simulink model "vienna_rectifier"  (R2026b)
settings: Solver=ode23tb  StopTime=param.sim.simlength  FixedStep=param.glb_time.tc  MaxStep=param.glb_time.tc
values from neighbouring files (symbols this model uses):
  param = struct()    [init_model.m]
undefined symbols (not defined in the file or in its folder): magnitude
libraries: fl_lib x42, nesl_utility x28, discrete_time_low_pass_filter x5, single_phase_transformer_lib x3, threephase_inductor_lib x1, dclink_for_three_levels x1, vienna_rectifier_ideal_switch_based_model x1, three_phase_three_levels_PWM_modulator x1, three_phase_voltage_with_frt_emulator x1
(part 2 of 4)

== system vienna_rectifier/grid/grid_emulator/3ph_Dyg ==
  Electrical Reference1 : fl_lib/Electrical/Electrical Elements/Electrical Reference
  ph1 : single_phase_transformer_lib/single phase transformer  Lm=param.grid.emu.trafo.Lm1 H  n1=param.grid.emu.trafo.n1  n2=param.grid.emu.trafo.n2  Rd1=param.grid.emu.trafo.Rd1 Ohm  Rd2=param.grid.emu.trafo.Rd2 Ohm  Ld1=param.grid.emu.trafo.Ld1 H  Ld2=param.grid.emu.trafo.Ld2 H  Rfe=param.grid.emu.trafo.Rfe1 Ohm  phi_specify=off  phi_priority=None  phi=0 V*s  phi_nominal_specify=off  phi_nominal_value=1  phi_nominal_unit=V*s  i1_specify=off  i1_priority=None  i1=0 A  i1_nominal_specify=off  i1_nominal_value=1  i1_nominal_unit=A  i2_specify=off  i2_priority=None  i2=0 A  i2_nominal_specify=off  i2_nominal_value=1  i2_nominal_unit=A  ife_specify=off  ife_priority=None  ife=0 A  ife_nominal_specify=off  ife_nominal_value=1  ife_nominal_unit=A  u1_specify=off  u1_priority=None  u1=0 V  u1_nominal_specify=off  u1_nominal_value=1  u1_nominal_unit=V  u2_specify=off  u2_priority=None  u2=0 V  u2_nominal_specify=off  u2_nominal_value=1  u2_nominal_unit=V
  ph2 : single_phase_transformer_lib/single phase transformer  Lm=param.grid.emu.trafo.Lm1 H  n1=param.grid.emu.trafo.n1  n2=param.grid.emu.trafo.n2  Rd1=param.grid.emu.trafo.Rd1 Ohm  Rd2=param.grid.emu.trafo.Rd2 Ohm  Ld1=param.grid.emu.trafo.Ld1 H  Ld2=param.grid.emu.trafo.Ld2 H  Rfe=param.grid.emu.trafo.Rfe1 Ohm  phi_specify=off  phi_priority=None  phi=0 V*s  phi_nominal_specify=off  phi_nominal_value=1  phi_nominal_unit=V*s  i1_specify=off  i1_priority=None  i1=0 A  i1_nominal_specify=off  i1_nominal_value=1  i1_nominal_unit=A  i2_specify=off  i2_priority=None  i2=0 A  i2_nominal_specify=off  i2_nominal_value=1  i2_nominal_unit=A  ife_specify=off  ife_priority=None  ife=0 A  ife_nominal_specify=off  ife_nominal_value=1  ife_nominal_unit=A  u1_specify=off  u1_priority=None  u1=0 V  u1_nominal_specify=off  u1_nominal_value=1  u1_nominal_unit=V  u2_specify=off  u2_priority=None  u2=0 V  u2_nominal_specify=off  u2_nominal_value=1  u2_nominal_unit=V
  ph3 : single_phase_transformer_lib/single phase transformer  Lm=param.grid.emu.trafo.Lm1 H  n1=param.grid.emu.trafo.n1  n2=param.grid.emu.trafo.n2  Rd1=param.grid.emu.trafo.Rd1 Ohm  Rd2=param.grid.emu.trafo.Rd2 Ohm  Ld1=param.grid.emu.trafo.Ld1 H  Ld2=param.grid.emu.trafo.Ld2 H  Rfe=param.grid.emu.trafo.Rfe1 Ohm  phi_specify=off  phi_priority=None  phi=0 V*s  phi_nominal_specify=off  phi_nominal_value=1  phi_nominal_unit=V*s  i1_specify=off  i1_priority=None  i1=0 A  i1_nominal_specify=off  i1_nominal_value=1  i1_nominal_unit=A  i2_specify=off  i2_priority=None  i2=0 A  i2_nominal_specify=off  i2_nominal_value=1  i2_nominal_unit=A  ife_specify=off  ife_priority=None  ife=0 A  ife_nominal_specify=off  ife_nominal_value=1  ife_nominal_unit=A  u1_specify=off  u1_priority=None  u1=0 V  u1_nominal_specify=off  u1_nominal_value=1  u1_nominal_unit=V  u2_specify=off  u2_priority=None  u2=0 V  u2_nominal_specify=off  u2_nominal_value=1  u2_nominal_unit=V
  ua : PMIOPort  Side=Right
  ub : PMIOPort  Port=2  Side=Right
  uc : PMIOPort  Port=3  Side=Right
  Ua : PMIOPort  Port=4  Side=Left
  Ub : PMIOPort  Port=5  Side=Left
  Uc : PMIOPort  Port=6  Side=Left
  connections:
  Electrical Reference1/LConn1 -- ph3/RConn2 -- ph2/RConn2 -- ph1/RConn2
  ph3/RConn1 -- uc/RConn1
  ph1/LConn1 -- ph3/LConn2 -- Ua/RConn1
  ph1/RConn1 -- ua/RConn1
  ph2/RConn1 -- ub/RConn1
  ph1/LConn2 -- ph2/LConn1 -- Ub/RConn1
  Uc/RConn1 -- ph3/LConn1 -- ph2/LConn2

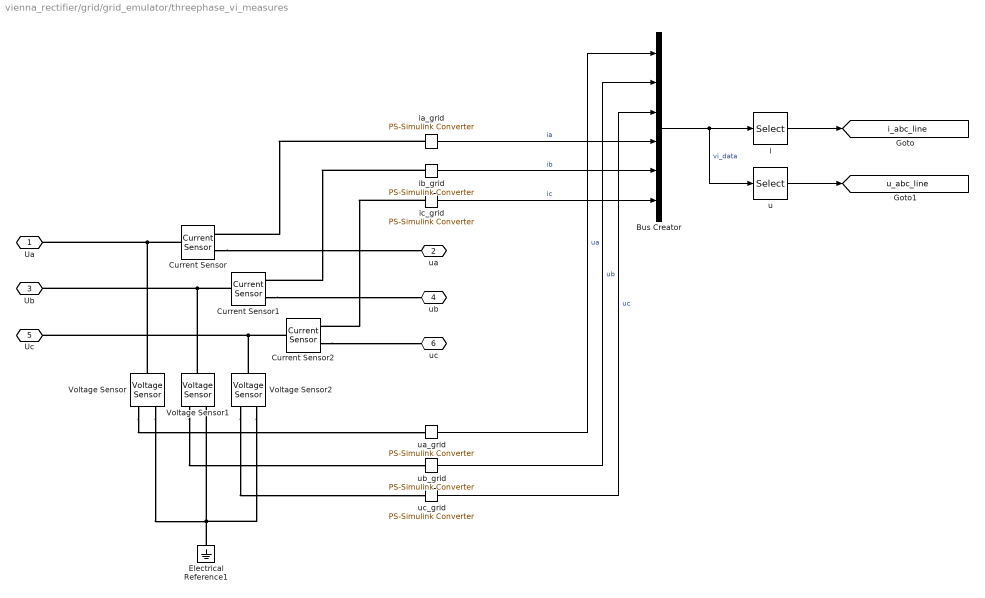
== system vienna_rectifier/grid/grid_emulator/threephase_vi_measures ==
  Bus Creator : BusCreator  Inputs=6
  Current Sensor : fl_lib/Electrical/Electrical Sensors/Current Sensor
  Current Sensor1 : fl_lib/Electrical/Electrical Sensors/Current Sensor
  Current Sensor2 : fl_lib/Electrical/Electrical Sensors/Current Sensor
  Electrical Reference1 : fl_lib/Electrical/Electrical Elements/Electrical Reference
  Voltage Sensor : fl_lib/Electrical/Electrical Sensors/Voltage Sensor
  Voltage Sensor1 : fl_lib/Electrical/Electrical Sensors/Voltage Sensor
  Voltage Sensor2 : fl_lib/Electrical/Electrical Sensors/Voltage Sensor
  i : Selector  InputPortWidth=6  IndexOptions=Index vector (dialog)  Indices=[4 5 6]  OutputSizes=1  RuntimeRangeChecks=off
  ia_grid : nesl_utility/PS-Simulink Converter  PhysicalDomain=network_engine_domain  SubClassName=ps_output  LeftPortType=input  RightPortType=output  PseudoPeriodic=off  Frequencies=[]  VectorFormat=1-D array  Unit=A  AffineConversion=off
  ib_grid : nesl_utility/PS-Simulink Converter  PhysicalDomain=network_engine_domain  SubClassName=ps_output  LeftPortType=input  RightPortType=output  PseudoPeriodic=off  Frequencies=[]  VectorFormat=1-D array  Unit=A  AffineConversion=off
  ic_grid : nesl_utility/PS-Simulink Converter  PhysicalDomain=network_engine_domain  SubClassName=ps_output  LeftPortType=input  RightPortType=output  PseudoPeriodic=off  Frequencies=[]  VectorFormat=1-D array  Unit=A  AffineConversion=off
  u : Selector  InputPortWidth=6  IndexOptions=Index vector (dialog)  Indices=[1 2 3]  OutputSizes=1  RuntimeRangeChecks=off
  ua_grid : nesl_utility/PS-Simulink Converter  PhysicalDomain=network_engine_domain  SubClassName=ps_output  LeftPortType=input  RightPortType=output  PseudoPeriodic=off  Frequencies=[]  VectorFormat=1-D array  Unit=V  AffineConversion=off
  ub_grid : nesl_utility/PS-Simulink Converter  PhysicalDomain=network_engine_domain  SubClassName=ps_output  LeftPortType=input  RightPortType=output  PseudoPeriodic=off  Frequencies=[]  VectorFormat=1-D array  Unit=V  AffineConversion=off
  uc_grid : nesl_utility/PS-Simulink Converter  PhysicalDomain=network_engine_domain  SubClassName=ps_output  LeftPortType=input  RightPortType=output  PseudoPeriodic=off  Frequencies=[]  VectorFormat=1-D array  Unit=V  AffineConversion=off
  Ua : PMIOPort  Side=Left
  ua : PMIOPort  Port=2  Side=Right
  Ub : PMIOPort  Port=3  Side=Left
  ub : PMIOPort  Port=4  Side=Right
  Uc : PMIOPort  Port=5  Side=Left
  uc : PMIOPort  Port=6  Side=Right
  tag scope: i_abc_line=global, u_abc_line=global
  wires:
  Bus Creator/1 -> i/1, u/1  "vi_data"
  ib_grid/1 -> Bus Creator/5  "ib"
  ia_grid/1 -> Bus Creator/4  "ia"
  ic_grid/1 -> Bus Creator/6  "ic"
  ua_grid/1 -> Bus Creator/1  "ua"
  ub_grid/1 -> Bus Creator/2  "ub"
  uc_grid/1 -> Bus Creator/3  "uc"
  i/1 -> [i_abc_line]
  u/1 -> [u_abc_line]
  connections:
  Current Sensor1/LConn1 -- Ub/RConn1 -- Voltage Sensor1/LConn1
  Electrical Reference1/LConn1 -- Voltage Sensor/RConn2 -- Voltage Sensor2/RConn2 -- Voltage Sensor1/RConn2
  Voltage Sensor/RConn1 -- ua_grid/LConn1
  Current Sensor/RConn2 -- ua/RConn1
  Voltage Sensor1/RConn1 -- ub_grid/LConn1
  Voltage Sensor2/LConn1 -- Current Sensor2/LConn1 -- Uc/RConn1
  Current Sensor/LConn1 -- Ua/RConn1 -- Voltage Sensor/LConn1
  Current Sensor1/RConn2 -- ub/RConn1
  Voltage Sensor2/RConn1 -- uc_grid/LConn1
  ib_grid/LConn1 -- Current Sensor1/RConn1
  ia_grid/LConn1 -- Current Sensor/RConn1
  ic_grid/LConn1 -- Current Sensor2/RConn1
  Current Sensor2/RConn2 -- uc/RConn1

== system vienna_rectifier/afe_dq_mod1/AFE_control/afe_control/acquisitions ==
  ug_abc_pu : Inport
  udc_pu : Inport  Port=2
  ig_abc_pu : Inport  Port=3
  is_abc_pu : Inport  Port=4
  master_time : Inport  Port=5
  grid_phase : Inport  Port=6
  Terminator : Terminator
  grid_phase_acquisition : Subsystem
  ig afe quantizzation and one step delay : Subsystem
  is afe quantizzation and one step delay : Subsystem
  phase_compensation_1 : Subsystem
  udc_acquisition : Subsystem
  ug afe quantizzation and one step delay : Subsystem
  AFE1_local_time_corr : Outport
  tag scope: grid_emulator_phase=scoped, igd_abc_pu=scoped, isd_abc_pu=scoped, udcd_pu_afe=scoped, ugd_abc_pu=scoped
  wires:
  grid_phase/1 -> grid_phase_acquisition/1(grid_phase)
  grid_phase_acquisition/1(grid_phased) -> [grid_emulator_phase]
  udc_acquisition/1(udcd_pu) -> [udcd_pu_afe]
  ig_abc_pu/1 -> ig afe quantizzation and one step delay/1(ig_abc_pu)
  ug_abc_pu/1 -> ug afe quantizzation and one step delay/1(ug_abc_pu)
  [udcd_pu_afe] -> Terminator/1
  phase_compensation_1/1(y) -> AFE1_local_time_corr/1
  is_abc_pu/1 -> is afe quantizzation and one step delay/1(is_abc_pu)
  master_time/1 -> phase_compensation_1/2(master_time)
  udc_pu/1 -> udc_acquisition/1(udc_pu)
  ig afe quantizzation and one step delay/1(igd_abc_pu) -> [igd_abc_pu]
  [local_time] -> phase_compensation_1/1(local_time)
  is afe quantizzation and one step delay/1(isd_abc_pu) -> [isd_abc_pu]
  ug afe quantizzation and one step delay/1(ugd_abc_pu) -> [ugd_abc_pu]

== system vienna_rectifier/afe_dq_mod1/AFE_control/afe_control/current_ctrl ==
  i_xi_ref : Inport
  Constant : Constant  Value=0
  Demux : Demux  Outputs=3
  current_transformation : Subsystem
  dq_vector_pi : Subsystem
  xi_eta_to_alpha_beta : MATLAB Function  TreatAsAtomicUnit=on
  zero_current_ctrl : Subsystem
  uabg : Outport  VectorParamsAs1DForOutWhenUnconnected=off
  wires:
  Demux/1 -> current_transformation/1(is_a_pu)  "is_a"
  Demux/2 -> current_transformation/2(is_b_pu)  "is_b"
  Demux/3 -> current_transformation/3(is_c_pu)  "is_c"
  [isd_abc_pu] -> Demux/1
  [phase_grid_pll] -> xi_eta_to_alpha_beta/3(phase)
  [id_xi_pu] -> dq_vector_pi/1(id)
  [id_eta_pu] -> dq_vector_pi/3(iq)
  i_xi_ref/1 -> dq_vector_pi/2(id_ref)
  Constant/1 -> dq_vector_pi/4(iq_ref)
  zero_current_ctrl/1(uabg_ctrl_out) -> uabg/1
  dq_vector_pi/1(md_sat) -> xi_eta_to_alpha_beta/1(xi)
  dq_vector_pi/2(mq_sat) -> xi_eta_to_alpha_beta/2(eta)
  xi_eta_to_alpha_beta/1(alpha) -> zero_current_ctrl/1(ualpha_ctrl_afe)
  xi_eta_to_alpha_beta/2(beta) -> zero_current_ctrl/2(ubeta_ctrl_afe)

== system vienna_rectifier/afe_dq_mod1/AFE_control/afe_control/data_to_worspace_module_1 ==
  Bus Creator : BusCreator  Inputs=3
  dq_pll : Subsystem
  pwr_meter : Subsystem
  m : Outport
  wires:
  Bus Creator/1 -> m/1
  pwr_meter/1(m_pwr_meter) -> Bus Creator/1  "pwr_meter"
  dq_pll/1(dqPLLs) -> Bus Creator/2  "dq_pll"
  [local_time] -> Bus Creator/3  "local_time"

== system vienna_rectifier/afe_dq_mod1/AFE_control/afe_control/grid_voltage_phase_lock_loops ==
  ug_abc_pu : Inport
  DDSRF-PLL : Subsystem
  tag scope: omega_grid_pll_pu=scoped, phase_grid_pll=scoped
  wires:
  ug_abc_pu/1 -> DDSRF-PLL/1(ug_abc_pu)
  DDSRF-PLL/1(gamma_grid_ddsrf_pll) -> [phase_grid_pll]
  DDSRF-PLL/2(omega_grid_ddsrf_pll) -> [omega_grid_pll_pu]

== system vienna_rectifier/afe_dq_mod1/AFE_control/afe_control/space_vector ==
  uab_out : Inport
  Bus Creator : BusCreator  Inputs=3
  Bus Selector : BusSelector  OutputSignals=da,db,dc
  Bus Selector1 : BusSelector  OutputSignals=ualpha_ctrl_afe,ubeta_ctrl_afe,ugamma_ctrl_afe
  C Caller : CCaller  FunctionName=sv_pwm_cm_process_simulink  PortSpecificationStruct="%)30     .    B H   8    (     @         %    \"     8    !     0         %  0 \"0    $    _    07)G3F%M90  4&]R=$YA;64 4V-O<&4     26YD97@     5'EP90      4VEZ90      27-';&]B86P   X    P    !@    @    $          4    (     0    ,    !         !   P!O=70 #@   #     &    \"     0         !0    @    !     P    $         $  # &]U=  .    .     8    (    !          %    \"     $    &     0         0   ...(+3252 chars)"
  Constant : Constant  Value=param.glb_time.ts_afe
  Constant1 : Constant
  Data Type Conversion1 : DataTypeConversion  OutDataTypeStr=double  SaturateOnIntegerOverflow=off  RndMeth=Floor
  Data Type Conversion{4,15..16,18} (4 alike) : DataTypeConversion  OutDataTypeStr=single  SaturateOnIntegerOverflow=off  RndMeth=Floor
  Data Type Conversion17 : DataTypeConversion  OutDataTypeStr=uint32  SaturateOnIntegerOverflow=off  RndMeth=Floor
  Data Type Conversion2 : DataTypeConversion  OutDataTypeStr=double  SaturateOnIntegerOverflow=off  RndMeth=Floor
  Data Type Conversion3 : DataTypeConversion  OutDataTypeStr=double  SaturateOnIntegerOverflow=off  RndMeth=Floor
  Gain1 : Gain  Gain=sqrt(3)/2
  Gain2 : Gain  Gain=sqrt(3)/2
  Gain3 : Gain  Gain=param.afe.behav.u_cm_comp_mod1
  duvw : Outport
  wires:
  Data Type Conversion15/1 -> C Caller/2
  Bus Selector/2 -> Data Type Conversion2/1  "<db>"
  Data Type Conversion18/1 -> C Caller/1
  C Caller/1 -> Bus Selector/1
  Bus Creator/1 -> duvw/1
  Data Type Conversion1/1 -> Bus Creator/1  "du(k)"
  Bus Selector1/2 -> Gain2/1  "<ubeta_ctrl_afe>"
  Bus Selector/3 -> Data Type Conversion3/1  "<dc>"
  Bus Selector1/1 -> Gain1/1  "<ualpha_ctrl_afe>"
  Data Type Conversion2/1 -> Bus Creator/2  "dv(k)"
  Gain2/1 -> Data Type Conversion15/1
  Bus Selector/1 -> Data Type Conversion1/1  "<da>"
  Gain1/1 -> Data Type Conversion18/1
  Data Type Conversion3/1 -> Bus Creator/3  "dw(k)"
  Constant/1 -> Data Type Conversion16/1
  uab_out/1 -> Bus Selector1/1
  Constant1/1 -> Data Type Conversion17/1
  Data Type Conversion16/1 -> C Caller/4
  Data Type Conversion17/1 -> C Caller/5
  Bus Selector1/3 -> Gain3/1  "<ugamma_ctrl_afe>"
  Gain3/1 -> Data Type Conversion4/1
  Data Type Conversion4/1 -> C Caller/3

== system vienna_rectifier/afe_dq_mod1/AFE_control/afe_control/udc_ctrl ==
  udc_pu : Inport
  1/Ti : Gain  Gain=param.afe.ctrl.kp_udc_ctrl  SaturateOnIntegerOverflow=on  OutDataTypeStr=Inherit: Same as input  ParamDataTypeStr=Inherit: Same as input
  Constant : Constant  Value=0
  Gain : Gain
  Saturation : Saturate  UpperLimit=param.afe.ctrl.ixi_pos_ref_lim  LowerLimit=-param.afe.ctrl.ixi_pos_ref_lim
  Sum1 : Sum  Inputs=+++  SaturateOnIntegerOverflow=on
  Sum2 : Sum  Inputs=-+  SaturateOnIntegerOverflow=on
  Sum3 : Sum  Inputs=-+  SaturateOnIntegerOverflow=on
  Switch : Switch  Criteria=u2 > Threshold  SaturateOnIntegerOverflow=off  InputSameDT=off
  To Workspace1 : ToWorkspace  VariableName=udc_pu_sim_mod1  SampleTime=-1
      settings: MaxDataPoints=param.glb_time.Ns_afe
  To Workspace3 : ToWorkspace  VariableName=udc_pu_ref_sim_mod1  SampleTime=-1
      settings: MaxDataPoints=param.glb_time.Ns_afe
  Unit Delay4 : UnitDelay  SampleTime=-1
  discrete-time-low-pass-filter1 : discrete_time_low_pass_filter/discrete-time-low-pass-filter  tau=20e-3  ts=param.glb_time.ts_afe
  kp : Gain  Gain=param.afe.ctrl.ki_udc_ctrl*param.glb_time.ts_afe  SaturateOnIntegerOverflow=on  OutDataTypeStr=Inherit: Same as input  ParamDataTypeStr=Inherit: Same as input
  pwr_lim_enable : Constant  Value=param.afe.behav.pwr_lim_enable
  udc_norm_ref : Step  Time=1e-3  FinalValue=param.afe.ctrl.udc_norm_ref
  udc_tracking : Scope  NumInputPorts=3
      settings: ActiveDisplayYMinimum=-0.20844726562499993  ActiveDisplayYMaximum=1.856494140625  DataLoggingVariableName=ScopeData8
  i_xi_ref : Outport
  wires:
  1/Ti/1 -> Sum1/1, Sum3/1
  kp/1 -> Sum1/2
  Sum3/1 -> Unit Delay4/1
  Unit Delay4/1 -> Sum1/3
  udc_norm_ref/1 -> discrete-time-low-pass-filter1/1
  udc_pu/1 -> Sum2/1, To Workspace1/1, udc_tracking/2  "udc_pu"
  Sum2/1 -> kp/1, 1/Ti/1
  Sum1/1 -> Saturation/1
  pwr_lim_enable/1 -> Switch/2
  Saturation/1 -> Switch/3
  Switch/1 -> Sum3/2, Gain/1
  Constant/1 -> Switch/1
  Gain/1 -> udc_tracking/3, i_xi_ref/1  "i_xi_ref"
  discrete-time-low-pass-filter1/1 -> To Workspace3/1, udc_tracking/1, Sum2/2  "udc_pu_ref"

== system vienna_rectifier/afe_dq_mod1/rectifier/deadtime_generator_for_ttype/dead_time_generator_cmos_simulink_phu ==
  gate_commands : Inport
  Bus Creator : BusCreator  Inputs=4
  Bus Selector : BusSelector  OutputSignals=gate_cmds_phu.cmd_gate_Q1,gate_cmds_phu.cmd_gate_Q4
  Bus Selector1 : BusSelector  OutputSignals=gate_cmds_phu.cmd_gate_Q2,gate_cmds_phu.cmd_gate_Q3
  Transfer Fcn{,1..3} (4 alike) : TransferFcn  Denominator=[ts 1]
  dead_time_leg_generator_1 : Subsystem  mask{Vpos_rail_dtg=positive_voltage_rail, deadtime=dead_time}
      mask prompts: Vpos_rail_dtg "Positive Voltage Rail Supply"; deadtime "DeadTime [s]"
  cmd_gates : Outport
  wires:
  Transfer Fcn1/1 -> dead_time_leg_generator_1/2(cmd_in_QB)  "gate_cmd_Q4"
  Transfer Fcn/1 -> dead_time_leg_generator_1/1(cmd_in_QA)  "gate_cmd_Q1"
  gate_commands/1 -> Bus Selector1/1, Bus Selector/1
  Bus Selector/1 -> Transfer Fcn/1  "<cmd_gate_Q1>"
  Bus Selector/2 -> Transfer Fcn1/1  "<cmd_gate_Q4>"
  Bus Selector1/1 -> Transfer Fcn2/1  "<cmd_gate_Q2>"
  Bus Selector1/2 -> Transfer Fcn3/1  "<cmd_gate_Q3>"
  dead_time_leg_generator_1/1(cmd_out_QA) -> [cmd_gate_Q1]  "cmd_gate_Q1"
  [cmd_gate_Q1] -> Bus Creator/1  "cmd_gate_Q1"
  Bus Creator/1 -> cmd_gates/1
  dead_time_leg_generator_1/2(cmd_out_QB) -> [cmd_gate_Q4]  "cmd_gate_Q4"
  Transfer Fcn3/1 -> [cmd_gate_Q3]  "cmd_gate_Q3"
  Transfer Fcn2/1 -> [cmd_gate_Q2]  "cmd_gate_Q2"
  [cmd_gate_Q2] -> Bus Creator/2  "cmd_gate_Q2"
  [cmd_gate_Q4] -> Bus Creator/4  "cmd_gate_Q4"
  [cmd_gate_Q3] -> Bus Creator/3  "cmd_gate_Q3"

== system vienna_rectifier/afe_dq_mod1/rectifier/deadtime_generator_for_ttype/dead_time_generator_cmos_simulink_phv ==
  gate_commands : Inport
  Bus Creator : BusCreator  Inputs=4
  Bus Selector : BusSelector  OutputSignals=gate_cmds_phv.cmd_gate_Q1,gate_cmds_phv.cmd_gate_Q4
  Bus Selector1 : BusSelector  OutputSignals=gate_cmds_phv.cmd_gate_Q2,gate_cmds_phv.cmd_gate_Q3
  Transfer Fcn{,1..3} (4 alike) : TransferFcn  Denominator=[ts 1]
  dead_time_leg_generator_1 : Subsystem  mask{Vpos_rail_dtg=positive_voltage_rail, deadtime=dead_time}
      mask prompts: Vpos_rail_dtg "Positive Voltage Rail Supply"; deadtime "DeadTime [s]"
  cmd_gates : Outport
  wires:
  [cmd_gate_Q3] -> Bus Creator/3  "cmd_gate_Q3"
  [cmd_gate_Q4] -> Bus Creator/4  "cmd_gate_Q4"
  [cmd_gate_Q2] -> Bus Creator/2  "cmd_gate_Q2"
  Transfer Fcn2/1 -> [cmd_gate_Q2]  "cmd_gate_Q2"
  Transfer Fcn3/1 -> [cmd_gate_Q3]  "cmd_gate_Q3"
  dead_time_leg_generator_1/2(cmd_out_QB) -> [cmd_gate_Q4]  "cmd_gate_Q4"
  Bus Creator/1 -> cmd_gates/1
  [cmd_gate_Q1] -> Bus Creator/1  "cmd_gate_Q1"
  dead_time_leg_generator_1/1(cmd_out_QA) -> [cmd_gate_Q1]  "cmd_gate_Q1"
  gate_commands/1 -> Bus Selector1/1, Bus Selector/1
  Transfer Fcn/1 -> dead_time_leg_generator_1/1(cmd_in_QA)  "gate_cmd_Q1"
  Transfer Fcn1/1 -> dead_time_leg_generator_1/2(cmd_in_QB)  "gate_cmd_Q4"
  Bus Selector/1 -> Transfer Fcn/1  "<cmd_gate_Q1>"
  Bus Selector/2 -> Transfer Fcn1/1  "<cmd_gate_Q4>"
  Bus Selector1/1 -> Transfer Fcn2/1  "<cmd_gate_Q2>"
  Bus Selector1/2 -> Transfer Fcn3/1  "<cmd_gate_Q3>"

== system vienna_rectifier/afe_dq_mod1/rectifier/deadtime_generator_for_ttype/dead_time_generator_cmos_simulink_phw ==
  gate_commands : Inport
  Bus Creator : BusCreator  Inputs=4
  Bus Selector : BusSelector  OutputSignals=gate_cmds_phw.cmd_gate_Q1,gate_cmds_phw.cmd_gate_Q4
  Bus Selector1 : BusSelector  OutputSignals=gate_cmds_phw.cmd_gate_Q2,gate_cmds_phw.cmd_gate_Q3
  Transfer Fcn{,1..3} (4 alike) : TransferFcn  Denominator=[ts 1]
  dead_time_leg_generator_1 : Subsystem  mask{Vpos_rail_dtg=positive_voltage_rail, deadtime=dead_time}
      mask prompts: Vpos_rail_dtg "Positive Voltage Rail Supply"; deadtime "DeadTime [s]"
  cmd_gates : Outport
  wires:
  Transfer Fcn1/1 -> dead_time_leg_generator_1/2(cmd_in_QB)  "gate_cmd_Q4"
  Transfer Fcn/1 -> dead_time_leg_generator_1/1(cmd_in_QA)  "gate_cmd_Q1"
  gate_commands/1 -> Bus Selector1/1, Bus Selector/1
  dead_time_leg_generator_1/1(cmd_out_QA) -> [cmd_gate_Q1]  "cmd_gate_Q1"
  [cmd_gate_Q1] -> Bus Creator/1  "cmd_gate_Q1"
  Bus Creator/1 -> cmd_gates/1
  dead_time_leg_generator_1/2(cmd_out_QB) -> [cmd_gate_Q4]  "cmd_gate_Q4"
  Transfer Fcn3/1 -> [cmd_gate_Q3]  "cmd_gate_Q3"
  Transfer Fcn2/1 -> [cmd_gate_Q2]  "cmd_gate_Q2"
  [cmd_gate_Q2] -> Bus Creator/2  "cmd_gate_Q2"
  [cmd_gate_Q4] -> Bus Creator/4  "cmd_gate_Q4"
  [cmd_gate_Q3] -> Bus Creator/3  "cmd_gate_Q3"
  Bus Selector/1 -> Transfer Fcn/1  "<cmd_gate_Q1>"
  Bus Selector/2 -> Transfer Fcn1/1  "<cmd_gate_Q4>"
  Bus Selector1/1 -> Transfer Fcn2/1  "<cmd_gate_Q2>"
  Bus Selector1/2 -> Transfer Fcn3/1  "<cmd_gate_Q3>"

== system vienna_rectifier/afe_dq_mod1/rectifier/sv_pwm/modulator1 ==
  u : Inport
  v : Inport  Port=2
  w : Inport  Port=3
  phase : Inport  Port=4
  Bus Creator : BusCreator  Inputs=3
  three_phase_three_levels_PWM_generator_with_global_TRGO1 : three_phase_three_levels_PWM_modulator/three_phase_three_levels_PWM_generator_with_global_TRGO1  f=param.glb_time.fPWM_AFE  m_up=1  m_low=-1  dead_time=0  pos_cmd_gate=15  neg_cmd_gate=0  polarity=1  tc=param.glb_time.tc  double_sampling=param.glb_time.TRGO_AFE_double_update
      link override gate commands/Bus Selector: OutputSignals=du(t)
      link override gate commands/Bus Selector1: OutputSignals=dv(t)
      link override gate commands/Bus Selector2: OutputSignals=dw(t)
  gate_cmds : Outport
  tag scope: TRGO_afe_module_1=global
  wires:
  [time_afe_module_1] -> three_phase_three_levels_PWM_generator_with_global_TRGO1/1
  Bus Creator/1 -> three_phase_three_levels_PWM_generator_with_global_TRGO1/3
  three_phase_three_levels_PWM_generator_with_global_TRGO1/1 -> [TRGO_afe_module_1]
  u/1 -> Bus Creator/1  "du(t)"
  v/1 -> Bus Creator/2  "dv(t)"
  w/1 -> Bus Creator/3  "dw(t)"
  phase/1 -> three_phase_three_levels_PWM_generator_with_global_TRGO1/2
  three_phase_three_levels_PWM_generator_with_global_TRGO1/2 -> gate_cmds/1

== system vienna_rectifier/afe_dq_mod1/AFE_control/afe_control/acquisitions/grid_phase_acquisition ==
  grid_phase : Inport
  Quantizer : Quantizer  QuantizationInterval=param.meas.adc_quantization
  Unit Delay : UnitDelay  SampleTime=-1
  Zero-Order Hold : ZeroOrderHold  SampleTime=-1
  grid_phased : Outport
  wires:
  Zero-Order Hold/1 -> Quantizer/1
  Unit Delay/1 -> grid_phased/1
  grid_phase/1 -> Zero-Order Hold/1
  Quantizer/1 -> Unit Delay/1

== system vienna_rectifier/afe_dq_mod1/AFE_control/afe_control/acquisitions/ig afe quantizzation and one step delay ==
  ig_abc_pu : Inport
  Demux1 : Demux  Outputs=3
  Mux1 : Mux  Inputs=3
  ig afe quantizzation and one step delay : Subsystem
  igd_abc_pu : Outport
  wires:
  Demux1/1 -> ig afe quantizzation and one step delay/1(ig_u_pu)
  Demux1/2 -> ig afe quantizzation and one step delay/2(ig_v_pu)
  ig_abc_pu/1 -> Demux1/1
  Mux1/1 -> igd_abc_pu/1
  Demux1/3 -> ig afe quantizzation and one step delay/3(ig_w_pu)
  ig afe quantizzation and one step delay/2(igd_v_pu) -> Mux1/2
  ig afe quantizzation and one step delay/1(igd_u_pu) -> Mux1/1
  ig afe quantizzation and one step delay/3(igd_w_pu) -> Mux1/3

== system vienna_rectifier/afe_dq_mod1/AFE_control/afe_control/acquisitions/is afe quantizzation and one step delay ==
  is_abc_pu : Inport
  Demux : Demux  Outputs=3
  Mux : Mux  Inputs=3
  is afe quantizzation and one step delay : Subsystem
  isd_abc_pu : Outport
  wires:
  is afe quantizzation and one step delay/2(isd_v_pu) -> Mux/2
  is_abc_pu/1 -> Demux/1
  is afe quantizzation and one step delay/3(isd_w_pu) -> Mux/3
  is afe quantizzation and one step delay/1(isd_u_pu) -> Mux/1
  Demux/1 -> is afe quantizzation and one step delay/1(is_u_pu)
  Mux/1 -> isd_abc_pu/1
  Demux/3 -> is afe quantizzation and one step delay/3(is_w_pu)
  Demux/2 -> is afe quantizzation and one step delay/2(is_v_pu)

== system vienna_rectifier/afe_dq_mod1/AFE_control/afe_control/acquisitions/phase_compensation_1 ==
  local_time : Inport
  master_time : Inport  Port=2
  Zero-Order Hold : ZeroOrderHold  SampleTime=-1
  Zero-Order Hold1 : ZeroOrderHold  SampleTime=-1
  alignment_eval_afe1 : Subsystem
  y : Outport
  wires:
  local_time/1 -> Zero-Order Hold/1
  master_time/1 -> Zero-Order Hold1/1
  alignment_eval_afe1/1(dp) -> y/1
  Zero-Order Hold/1 -> alignment_eval_afe1/1(local_time)
  Zero-Order Hold1/1 -> alignment_eval_afe1/2(master_time)

== system vienna_rectifier/afe_dq_mod1/AFE_control/afe_control/acquisitions/udc_acquisition ==
  udc_pu : Inport
  Quantizer : Quantizer  QuantizationInterval=param.meas.adc_quantization
  Unit Delay : UnitDelay  SampleTime=-1
  Zero-Order Hold : ZeroOrderHold  SampleTime=-1
  udcd_pu : Outport
  wires:
  Quantizer/1 -> Unit Delay/1
  udc_pu/1 -> Zero-Order Hold/1
  Unit Delay/1 -> udcd_pu/1
  Zero-Order Hold/1 -> Quantizer/1

== system vienna_rectifier/afe_dq_mod1/AFE_control/afe_control/acquisitions/ug afe quantizzation and one step delay ==
  ug_abc_pu : Inport
  Demux : Demux  Outputs=3
  Mux : Mux  Inputs=3
  ug afe quantizzation and one step delay : Subsystem
  ugd_abc_pu : Outport
  wires:
  ug afe quantizzation and one step delay/2(ugd_v_pu) -> Mux/2
  Demux/2 -> ug afe quantizzation and one step delay/2(ug_v_pu)
  Demux/3 -> ug afe quantizzation and one step delay/3(ug_w_pu)
  ug afe quantizzation and one step delay/1(ugd_u_pu) -> Mux/1
  Demux/1 -> ug afe quantizzation and one step delay/1(ug_u_pu)
  ug_abc_pu/1 -> Demux/1
  ug afe quantizzation and one step delay/3(ugd_w_pu) -> Mux/3
  Mux/1 -> ugd_abc_pu/1

== system vienna_rectifier/afe_dq_mod1/AFE_control/afe_control/current_ctrl/current_transformation ==
  is_a_pu : Inport
  is_b_pu : Inport  Port=2
  is_c_pu : Inport  Port=3
  alphabeta2xieta : MATLAB Function  TreatAsAtomicUnit=on
  uvw2alphabeta : MATLAB Function  TreatAsAtomicUnit=on
  tag scope: id_eta_pu=scoped, id_xi_pu=scoped
  wires:
  is_c_pu/1 -> uvw2alphabeta/3(w)
  alphabeta2xieta/2(eta) -> [id_eta_pu]  "ieta_pu"
  alphabeta2xieta/1(xi) -> [id_xi_pu]  "ixi_pu"
  is_b_pu/1 -> uvw2alphabeta/2(v)
  uvw2alphabeta/2(beta) -> alphabeta2xieta/2(beta)  "ibeta_pu"
  uvw2alphabeta/1(alpha) -> alphabeta2xieta/1(alpha)  "ialpha_pu"
  [phase_grid_pll] -> alphabeta2xieta/3(gamma)
  is_a_pu/1 -> uvw2alphabeta/1(u)

== system vienna_rectifier/afe_dq_mod1/AFE_control/afe_control/current_ctrl/dq_vector_pi ==
  id : Inport
  id_ref : Inport  Port=2
  iq : Inport  Port=3
  iq_ref : Inport  Port=4
  Sum1 : Sum  Inputs=|-+
  Sum2 : Sum  Inputs=|-+
  bounder1 : Subsystem
  bounder2 : Subsystem
  pi_d : Subsystem
  pi_q : Subsystem
  switch : Subsystem
  vector lenght : Subsystem
  md_sat : Outport
  mq_sat : Outport  Port=2
  wires:
  bounder2/2(clip) -> switch/2(clip 2)
  vector lenght/2(m) -> bounder1/3(m), bounder2/1(m)
  Sum2/1 -> pi_q/1(iq_tilde)
  pi_d/1(ud_out) -> vector lenght/1(md), bounder1/1(md)
  pi_q/1(Vqs_out) -> bounder2/3(mq), vector lenght/2(mq)
  vector lenght/1(m_1) -> bounder1/2(m_1), bounder2/2(m_1)
  switch/1(clip) -> pi_q/2(clip), pi_d/2(clip)
  iq/1 -> Sum2/1
  Sum1/1 -> pi_d/1(id_tilde)
  bounder1/2(clip) -> switch/1(clip 1)
  id/1 -> Sum1/1
  bounder1/1(md_sat) -> md_sat/1
  bounder2/1(mq_sat) -> mq_sat/1
  id_ref/1 -> Sum1/2
  iq_ref/1 -> Sum2/2

== system vienna_rectifier/afe_dq_mod1/AFE_control/afe_control/current_ctrl/zero_current_ctrl ==
  ualpha_ctrl_afe : Inport
  ubeta_ctrl_afe : Inport  Port=2
  Bus Creator1 : BusCreator  Inputs=3
  iz : Subsystem
  zero_sequence_current_ctrl : Subsystem
  uabg_ctrl_out : Outport
  wires:
  Bus Creator1/1 -> uabg_ctrl_out/1
  ualpha_ctrl_afe/1 -> Bus Creator1/1  "ualpha_ctrl_afe"
  ubeta_ctrl_afe/1 -> Bus Creator1/2  "ubeta_ctrl_afe"
  iz/1(iz) -> zero_sequence_current_ctrl/1(iz)
  zero_sequence_current_ctrl/1(ugamma_afe) -> Bus Creator1/3  "ugamma_ctrl_afe"

== system vienna_rectifier/afe_dq_mod1/AFE_control/afe_control/data_to_worspace_module_1/dq_pll ==
  Bus Creator1 : BusCreator  Inputs=8
  From1 : From  Commented=on  GotoTag=phase_grid_fht_simulink_pll
  From13 : From  Commented=on  GotoTag=phase_grid_dqpll_ccaller
  From14 : From  Commented=on  GotoTag=omega_grid_dqpll_ccaller
  From19 : From  Commented=on  GotoTag=phase_grid_fhtsr_dqpll
  From2 : From  Commented=on  GotoTag=omega_grid_fht_simulink_pll
  From20 : From  Commented=on  GotoTag=omega_grid_fhtsr_dqpll
  dqPLLs : Outport
  wires:
  From1/1 -> Bus Creator1/5  "phase_grid_fht_simulink_pll"
  From2/1 -> Bus Creator1/6  "omega_grid_fht_simulink_pll"
  From20/1 -> Bus Creator1/8  "omega_grid_fhtsr_dqpll"
  From19/1 -> Bus Creator1/7  "phase_grid_fhtsr_dqpll"
  From14/1 -> Bus Creator1/4  "omega_grid_dqpll_ccaller"
  From13/1 -> Bus Creator1/3  "phase_grid_dqpll_ccaller"
  [omega_grid_pll_pu] -> Bus Creator1/2  "omega_grid_pll_pu"
  [phase_grid_pll] -> Bus Creator1/1  "phase_grid_pll"
  Bus Creator1/1 -> dqPLLs/1

== system vienna_rectifier/afe_dq_mod1/AFE_control/afe_control/data_to_worspace_module_1/pwr_meter ==
  Bus Creator1 : BusCreator  Inputs=4
  From : From  Commented=on  GotoTag=pwr_act_grid
  From1 : From  Commented=on  GotoTag=i_grid_pu_rms
  From2 : From  Commented=on  GotoTag=u_grid_pu_rms
  From6 : From  Commented=on  GotoTag=pwr_react_grid
  m_pwr_meter : Outport
  wires:
  From2/1 -> Bus Creator1/2  "u_grid_pu_rms"
  Bus Creator1/1 -> m_pwr_meter/1
  From/1 -> Bus Creator1/3  "pwr_act_grid"
  From6/1 -> Bus Creator1/4  "pwr_react_grid"
  From1/1 -> Bus Creator1/1  "i_grid_pu_rms"

== system vienna_rectifier/afe_dq_mod1/AFE_control/afe_control/grid_voltage_phase_lock_loops/DDSRF-PLL ==
  ug_abc_pu : Inport
  pll_stageA : Subsystem
  pll_stageB : Subsystem
  gamma_grid_ddsrf_pll : Outport
  omega_grid_ddsrf_pll : Outport  Port=2
  wires:
  pll_stageB/1(phase_grid_ddsrf_pll) -> pll_stageA/1(gamma_grid), gamma_grid_ddsrf_pll/1
  pll_stageA/2(u_grid_pos_eta) -> pll_stageB/2(u_grid_pos_eta)  "u_grid_pos_eta"
  pll_stageA/1(u_grid_pos_xi) -> pll_stageB/1(u_grid_pos_xi)  "u_grid_pos_xi"
  pll_stageB/2(omega_grid_ddsrf_pll) -> omega_grid_ddsrf_pll/1
  ug_abc_pu/1 -> pll_stageA/2(ug_abc_pu)

== system vienna_rectifier/afe_dq_mod1/rectifier/deadtime_generator_for_ttype/dead_time_generator_cmos_simulink_phu/dead_time_leg_generator_1 ==
  cmd_in_QA : Inport
  cmd_in_QB : Inport  Port=2
  MATLAB Function : MATLAB Function  TreatAsAtomicUnit=on
  MATLAB Function1 : MATLAB Function  TreatAsAtomicUnit=on
  MATLAB Function2 : MATLAB Function  TreatAsAtomicUnit=on
  MATLAB Function3 : MATLAB Function  TreatAsAtomicUnit=on
  MATLAB Function4 : MATLAB Function  TreatAsAtomicUnit=on
  MATLAB Function5 : MATLAB Function  TreatAsAtomicUnit=on
  MATLAB Function6 : MATLAB Function  TreatAsAtomicUnit=on
  MATLAB Function7 : MATLAB Function  TreatAsAtomicUnit=on
  MATLAB Function8 : MATLAB Function  TreatAsAtomicUnit=on
  MATLAB Function9 : MATLAB Function  TreatAsAtomicUnit=on
  Transfer Fcn : TransferFcn  Denominator=[sqrt(2)*deadtime 1]
  Transfer Fcn1 : TransferFcn  Denominator=[sqrt(2)*deadtime 1]
  cmd_out_QA : Outport
  cmd_out_QB : Outport  Port=2
  wires:
  MATLAB Function8/1(y) -> MATLAB Function5/2(u2)
  MATLAB Function7/1(y) -> Transfer Fcn1/1, MATLAB Function9/2(u2)
  MATLAB Function3/1(y) -> MATLAB Function1/2(u2)
  MATLAB Function2/1(y) -> Transfer Fcn/1, MATLAB Function4/1(u1)
  MATLAB Function/1(y) -> MATLAB Function1/1(u1), MATLAB Function2/1(u)
  MATLAB Function9/1(y) -> cmd_out_QB/1
  MATLAB Function4/1(y) -> cmd_out_QA/1
  MATLAB Function6/1(y) -> MATLAB Function5/1(u1), MATLAB Function7/1(u)
  cmd_in_QA/1 -> MATLAB Function/1(u)
  MATLAB Function5/1(y) -> MATLAB Function4/2(u2)
  MATLAB Function1/1(y) -> MATLAB Function9/1(u1)
  cmd_in_QB/1 -> MATLAB Function6/1(u)
  Transfer Fcn1/1 -> MATLAB Function8/1(u)
  Transfer Fcn/1 -> MATLAB Function3/1(u)

== system vienna_rectifier/afe_dq_mod1/rectifier/deadtime_generator_for_ttype/dead_time_generator_cmos_simulink_phv/dead_time_leg_generator_1 ==
  cmd_in_QA : Inport
  cmd_in_QB : Inport  Port=2
  MATLAB Function : MATLAB Function  TreatAsAtomicUnit=on
  MATLAB Function1 : MATLAB Function  TreatAsAtomicUnit=on
  MATLAB Function2 : MATLAB Function  TreatAsAtomicUnit=on
  MATLAB Function3 : MATLAB Function  TreatAsAtomicUnit=on
  MATLAB Function4 : MATLAB Function  TreatAsAtomicUnit=on
  MATLAB Function5 : MATLAB Function  TreatAsAtomicUnit=on
  MATLAB Function6 : MATLAB Function  TreatAsAtomicUnit=on
  MATLAB Function7 : MATLAB Function  TreatAsAtomicUnit=on
  MATLAB Function8 : MATLAB Function  TreatAsAtomicUnit=on
  MATLAB Function9 : MATLAB Function  TreatAsAtomicUnit=on
  Transfer Fcn : TransferFcn  Denominator=[sqrt(2)*deadtime 1]
  Transfer Fcn1 : TransferFcn  Denominator=[sqrt(2)*deadtime 1]
  cmd_out_QA : Outport
  cmd_out_QB : Outport  Port=2
  wires:
  Transfer Fcn/1 -> MATLAB Function3/1(u)
  Transfer Fcn1/1 -> MATLAB Function8/1(u)
  cmd_in_QB/1 -> MATLAB Function6/1(u)
  MATLAB Function1/1(y) -> MATLAB Function9/1(u1)
  MATLAB Function5/1(y) -> MATLAB Function4/2(u2)
  cmd_in_QA/1 -> MATLAB Function/1(u)
  MATLAB Function6/1(y) -> MATLAB Function7/1(u), MATLAB Function5/1(u1)
  MATLAB Function4/1(y) -> cmd_out_QA/1
  MATLAB Function9/1(y) -> cmd_out_QB/1
  MATLAB Function/1(y) -> MATLAB Function2/1(u), MATLAB Function1/1(u1)
  MATLAB Function2/1(y) -> MATLAB Function4/1(u1), Transfer Fcn/1
  MATLAB Function3/1(y) -> MATLAB Function1/2(u2)
  MATLAB Function7/1(y) -> MATLAB Function9/2(u2), Transfer Fcn1/1
  MATLAB Function8/1(y) -> MATLAB Function5/2(u2)

== system vienna_rectifier/afe_dq_mod1/rectifier/deadtime_generator_for_ttype/dead_time_generator_cmos_simulink_phw/dead_time_leg_generator_1 ==
  cmd_in_QA : Inport
  cmd_in_QB : Inport  Port=2
  MATLAB Function : MATLAB Function  TreatAsAtomicUnit=on
  MATLAB Function1 : MATLAB Function  TreatAsAtomicUnit=on
  MATLAB Function2 : MATLAB Function  TreatAsAtomicUnit=on
  MATLAB Function3 : MATLAB Function  TreatAsAtomicUnit=on
  MATLAB Function4 : MATLAB Function  TreatAsAtomicUnit=on
  MATLAB Function5 : MATLAB Function  TreatAsAtomicUnit=on
  MATLAB Function6 : MATLAB Function  TreatAsAtomicUnit=on
  MATLAB Function7 : MATLAB Function  TreatAsAtomicUnit=on
  MATLAB Function8 : MATLAB Function  TreatAsAtomicUnit=on
  MATLAB Function9 : MATLAB Function  TreatAsAtomicUnit=on
  Transfer Fcn : TransferFcn  Denominator=[sqrt(2)*deadtime 1]
  Transfer Fcn1 : TransferFcn  Denominator=[sqrt(2)*deadtime 1]
  cmd_out_QA : Outport
  cmd_out_QB : Outport  Port=2
  wires:
  MATLAB Function8/1(y) -> MATLAB Function5/2(u2)
  MATLAB Function7/1(y) -> Transfer Fcn1/1, MATLAB Function9/2(u2)
  MATLAB Function3/1(y) -> MATLAB Function1/2(u2)
  MATLAB Function2/1(y) -> Transfer Fcn/1, MATLAB Function4/1(u1)
  MATLAB Function/1(y) -> MATLAB Function1/1(u1), MATLAB Function2/1(u)
  MATLAB Function9/1(y) -> cmd_out_QB/1
  MATLAB Function4/1(y) -> cmd_out_QA/1
  MATLAB Function6/1(y) -> MATLAB Function5/1(u1), MATLAB Function7/1(u)
  cmd_in_QA/1 -> MATLAB Function/1(u)
  MATLAB Function5/1(y) -> MATLAB Function4/2(u2)
  MATLAB Function1/1(y) -> MATLAB Function9/1(u1)
  cmd_in_QB/1 -> MATLAB Function6/1(u)
  Transfer Fcn1/1 -> MATLAB Function8/1(u)
  Transfer Fcn/1 -> MATLAB Function3/1(u)

== system vienna_rectifier/afe_dq_mod1/AFE_control/afe_control/acquisitions/ig afe quantizzation and one step delay/ig afe quantizzation and one step delay ==
  ig_u_pu : Inport
  ig_v_pu : Inport  Port=2
  ig_w_pu : Inport  Port=3
  Gain4 : Gain  Gain=-1
  Gain5 : Gain  Gain=-1
  Gain6 : Gain  Gain=-1
  Quantizer1 : Quantizer  QuantizationInterval=param.meas.adc_quantization
  Quantizer2 : Quantizer  QuantizationInterval=param.meas.adc_quantization
  Quantizer4 : Quantizer  QuantizationInterval=param.meas.adc_quantization
  Unit Delay : UnitDelay  SampleTime=-1
  Unit Delay1 : UnitDelay  SampleTime=-1
  Unit Delay2 : UnitDelay  SampleTime=-1
  Zero-Order Hold : ZeroOrderHold  SampleTime=-1
  Zero-Order Hold1 : ZeroOrderHold  SampleTime=-1
  Zero-Order Hold2 : ZeroOrderHold  SampleTime=-1
  igd_u_pu : Outport
  igd_v_pu : Outport  Port=2
  igd_w_pu : Outport  Port=3
  wires:
  Quantizer1/1 -> Unit Delay1/1
  Quantizer4/1 -> Unit Delay/1
  Quantizer2/1 -> Unit Delay2/1
  ig_u_pu/1 -> Zero-Order Hold/1
  ig_v_pu/1 -> Zero-Order Hold1/1
  ig_w_pu/1 -> Zero-Order Hold2/1
  Unit Delay/1 -> Gain4/1
  Unit Delay1/1 -> Gain5/1
  Unit Delay2/1 -> Gain6/1
  Gain4/1 -> igd_u_pu/1
  Gain5/1 -> igd_v_pu/1
  Gain6/1 -> igd_w_pu/1
  Zero-Order Hold/1 -> Quantizer4/1
  Zero-Order Hold1/1 -> Quantizer1/1
  Zero-Order Hold2/1 -> Quantizer2/1

== system vienna_rectifier/afe_dq_mod1/AFE_control/afe_control/acquisitions/is afe quantizzation and one step delay/is afe quantizzation and one step delay ==
  is_u_pu : Inport
  is_v_pu : Inport  Port=2
  is_w_pu : Inport  Port=3
  Gain : Gain  Gain=-1
  Gain1 : Gain  Gain=-1
  Gain2 : Gain  Gain=-1
  Quantizer : Quantizer  QuantizationInterval=param.meas.adc_quantization
  Quantizer1 : Quantizer  QuantizationInterval=param.meas.adc_quantization
  Quantizer2 : Quantizer  QuantizationInterval=param.meas.adc_quantization
  Unit Delay : UnitDelay  SampleTime=-1
  Unit Delay1 : UnitDelay  SampleTime=-1
  Unit Delay2 : UnitDelay  SampleTime=-1
  Zero-Order Hold : ZeroOrderHold  SampleTime=-1
  Zero-Order Hold1 : ZeroOrderHold  SampleTime=-1
  Zero-Order Hold2 : ZeroOrderHold  SampleTime=-1
  isd_u_pu : Outport
  isd_v_pu : Outport  Port=2
  isd_w_pu : Outport  Port=3
  wires:
  Unit Delay/1 -> Gain/1
  Unit Delay1/1 -> Gain1/1
  Unit Delay2/1 -> Gain2/1
  Quantizer/1 -> Unit Delay/1
  Quantizer1/1 -> Unit Delay1/1
  Quantizer2/1 -> Unit Delay2/1
  is_u_pu/1 -> Zero-Order Hold/1
  is_v_pu/1 -> Zero-Order Hold1/1
  is_w_pu/1 -> Zero-Order Hold2/1
  Zero-Order Hold/1 -> Quantizer/1
  Zero-Order Hold1/1 -> Quantizer1/1
  Zero-Order Hold2/1 -> Quantizer2/1
  Gain/1 -> isd_u_pu/1
  Gain1/1 -> isd_v_pu/1
  Gain2/1 -> isd_w_pu/1

== system vienna_rectifier/afe_dq_mod1/AFE_control/afe_control/acquisitions/phase_compensation_1/alignment_eval_afe1 ==
  local_time : Inport
  master_time : Inport  Port=2
  Constant : Constant  Value=0
  Gain : Gain  Gain=-1
  Sum : Sum  Inputs=|+-
  pi : Subsystem  mask{kp=param.ctrl.align.kp, ki=param.ctrl.align.ki*param.glb_time.ts_afe, lim_up=param.ctrl.align.lim_up, lim_down=param.ctrl.align.lim_down}
      mask prompts: ki "ki*ts"
      mask Display:
      | disp('pi()');
      | port_label('input', 1, 'u_ref');
      | port_label('input', 2, 'u');
      | port_label('output', 1, 'y');
  dp : Outport
  wires:
  master_time/1 -> Sum/1
  Sum/1 -> Gain/1
  Constant/1 -> pi/1(u_ref)
  local_time/1 -> Sum/2
  Gain/1 -> pi/2(u)
  pi/1(y) -> dp/1

== system vienna_rectifier/afe_dq_mod1/AFE_control/afe_control/acquisitions/ug afe quantizzation and one step delay/ug afe quantizzation and one step delay ==
  ug_u_pu : Inport
  ug_v_pu : Inport  Port=2
  ug_w_pu : Inport  Port=3
  Quantizer1 : Quantizer  QuantizationInterval=param.meas.adc_quantization
  Quantizer2 : Quantizer  QuantizationInterval=param.meas.adc_quantization
  Quantizer4 : Quantizer  QuantizationInterval=param.meas.adc_quantization
  Unit Delay : UnitDelay  SampleTime=-1
  Unit Delay1 : UnitDelay  SampleTime=-1
  Unit Delay2 : UnitDelay  SampleTime=-1
  Zero-Order Hold : ZeroOrderHold  SampleTime=-1
  Zero-Order Hold1 : ZeroOrderHold  SampleTime=-1
  Zero-Order Hold2 : ZeroOrderHold  SampleTime=-1
  ugd_u_pu : Outport
  ugd_v_pu : Outport  Port=2
  ugd_w_pu : Outport  Port=3
  wires:
  Unit Delay/1 -> ugd_u_pu/1
  Unit Delay1/1 -> ugd_v_pu/1
  Unit Delay2/1 -> ugd_w_pu/1
  Quantizer4/1 -> Unit Delay/1
  Quantizer1/1 -> Unit Delay1/1
  Quantizer2/1 -> Unit Delay2/1
  ug_w_pu/1 -> Zero-Order Hold2/1
  ug_v_pu/1 -> Zero-Order Hold1/1
  ug_u_pu/1 -> Zero-Order Hold/1
  Zero-Order Hold/1 -> Quantizer4/1
  Zero-Order Hold1/1 -> Quantizer1/1
  Zero-Order Hold2/1 -> Quantizer2/1

== system vienna_rectifier/afe_dq_mod1/AFE_control/afe_control/current_ctrl/dq_vector_pi/bounder1 ==
  md : Inport
  m_1 : Inport  Port=2
  m : Inport  Port=3
  Constant : Constant
  Constant1 : Constant  Value=0
  Divide : Product
  Switch : Switch  Threshold=1  SaturateOnIntegerOverflow=off  InputSameDT=off
  Switch1 : Switch  Threshold=1  SaturateOnIntegerOverflow=off  InputSameDT=off
  md_sat : Outport  VectorParamsAs1DForOutWhenUnconnected=off
  clip : Outport  Port=2  VectorParamsAs1DForOutWhenUnconnected=off
  wires:
  md/1 -> Switch1/3, Divide/2
  m_1/1 -> Divide/1
  Divide/1 -> Switch1/1
  Switch1/1 -> md_sat/1
  Switch/1 -> clip/1
  m/1 -> Switch/2, Switch1/2
  Constant/1 -> Switch/1
  Constant1/1 -> Switch/3

== system vienna_rectifier/afe_dq_mod1/AFE_control/afe_control/current_ctrl/dq_vector_pi/bounder2 ==
  m : Inport
  m_1 : Inport  Port=2
  mq : Inport  Port=3
  Constant : Constant
  Constant1 : Constant  Value=0
  Divide : Product
  Switch : Switch  Threshold=1  SaturateOnIntegerOverflow=off  InputSameDT=off
  Switch1 : Switch  Threshold=1  SaturateOnIntegerOverflow=off  InputSameDT=off
  mq_sat : Outport  VectorParamsAs1DForOutWhenUnconnected=off
  clip : Outport  Port=2  VectorParamsAs1DForOutWhenUnconnected=off
  wires:
  Constant1/1 -> Switch/3
  Constant/1 -> Switch/1
  m/1 -> Switch1/2, Switch/2
  Switch/1 -> clip/1
  Switch1/1 -> mq_sat/1
  Divide/1 -> Switch1/1
  m_1/1 -> Divide/1
  mq/1 -> Divide/2, Switch1/3

== system vienna_rectifier/afe_dq_mod1/AFE_control/afe_control/current_ctrl/dq_vector_pi/pi_d ==
  id_tilde : Inport
  clip : Inport  Port=2
  1/Ti : Gain  Gain=param.afe.ctrl.kp_is_xi  SaturateOnIntegerOverflow=on  OutDataTypeStr=Inherit: Same as input  ParamDataTypeStr=Inherit: Same as input
  Constant : Constant  Value=0
  Sum2 : Sum  Inputs=+-  SaturateOnIntegerOverflow=on
  Sum4 : Sum  SaturateOnIntegerOverflow=on
  Sum5 : Sum  SaturateOnIntegerOverflow=on
  Switch1 : Switch  Threshold=0.5  SaturateOnIntegerOverflow=off  InputSameDT=off
  Switch2 : Switch  Threshold=0.5  SaturateOnIntegerOverflow=off  InputSameDT=off
  Unit Delay1 : UnitDelay  SampleTime=-1
  Unit Delay2 : UnitDelay  SampleTime=-1
  kp1 : Gain  Gain=param.ctrl.clip_release*param.glb_time.ts_afe  SaturateOnIntegerOverflow=on  OutDataTypeStr=Inherit: Same as input  ParamDataTypeStr=Inherit: Same as input
  kp2 : Gain  Gain=param.afe.ctrl.ki_is_xi*param.glb_time.ts_afe  SaturateOnIntegerOverflow=on  OutDataTypeStr=Inherit: Same as input  ParamDataTypeStr=Inherit: Same as input
  ud_out : Outport  VectorParamsAs1DForOutWhenUnconnected=off
  wires:
  id_tilde/1 -> kp2/1, 1/Ti/1
  Sum5/1 -> ud_out/1
  Switch1/1 -> Unit Delay2/1
  Sum4/1 -> Sum5/2, Switch1/3
  kp1/1 -> Sum2/2
  Sum2/1 -> Switch1/1
  Unit Delay2/1 -> Sum4/2, kp1/1, Sum2/1
  1/Ti/1 -> Sum5/1
  Switch2/1 -> Sum4/1
  kp2/1 -> Switch2/3
  clip/1 -> Unit Delay1/1
  [clip] -> Switch2/2
  [clip] -> Switch1/2
  Constant/1 -> Switch2/1
  Unit Delay1/1 -> [clip]

== system vienna_rectifier/afe_dq_mod1/AFE_control/afe_control/current_ctrl/dq_vector_pi/pi_q ==
  iq_tilde : Inport
  clip : Inport  Port=2
  1/Ti : Gain  Gain=param.afe.ctrl.kp_is_eta  SaturateOnIntegerOverflow=on  OutDataTypeStr=Inherit: Same as input  ParamDataTypeStr=Inherit: Same as input
  Constant : Constant  Value=0
  Sum2 : Sum  Inputs=+-  SaturateOnIntegerOverflow=on
  Sum4 : Sum  SaturateOnIntegerOverflow=on
  Sum5 : Sum  SaturateOnIntegerOverflow=on
  Switch1 : Switch  Threshold=0.5  SaturateOnIntegerOverflow=off  InputSameDT=off
  Switch2 : Switch  Threshold=0.5  SaturateOnIntegerOverflow=off  InputSameDT=off
  Unit Delay1 : UnitDelay  SampleTime=-1
  Unit Delay2 : UnitDelay  SampleTime=-1
  kp1 : Gain  Gain=param.ctrl.clip_release*param.glb_time.ts_afe  SaturateOnIntegerOverflow=on  OutDataTypeStr=Inherit: Same as input  ParamDataTypeStr=Inherit: Same as input
  kp2 : Gain  Gain=param.afe.ctrl.ki_is_eta*param.glb_time.ts_afe  SaturateOnIntegerOverflow=on  OutDataTypeStr=Inherit: Same as input  ParamDataTypeStr=Inherit: Same as input
  Vqs_out : Outport  VectorParamsAs1DForOutWhenUnconnected=off
  wires:
  Constant/1 -> Switch2/1
  [clip] -> Switch1/2
  [clip] -> Switch2/2
  clip/1 -> Unit Delay1/1
  kp2/1 -> Switch2/3
  Switch2/1 -> Sum4/1
  1/Ti/1 -> Sum5/1
  Unit Delay2/1 -> Sum2/1, kp1/1, Sum4/2
  Sum2/1 -> Switch1/1
  kp1/1 -> Sum2/2
  Sum4/1 -> Sum5/2, Switch1/3
  Switch1/1 -> Unit Delay2/1
  iq_tilde/1 -> 1/Ti/1, kp2/1
  Unit Delay1/1 -> [clip]
  Sum5/1 -> Vqs_out/1

== system vienna_rectifier/afe_dq_mod1/AFE_control/afe_control/current_ctrl/dq_vector_pi/switch ==
  clip 1 : Inport
  clip 2 : Inport  Port=2
  Constant4 : Constant
  Constant5 : Constant  Value=0
  Sum1 : Sum  SaturateOnIntegerOverflow=on
  Switch : Switch  Threshold=0.5  SaturateOnIntegerOverflow=off  InputSameDT=off
  clip : Outport  VectorParamsAs1DForOutWhenUnconnected=off
  wires:
  Constant5/1 -> Switch/3
  Switch/1 -> clip/1
  Constant4/1 -> Switch/1
  Sum1/1 -> Switch/2
  clip 1/1 -> Sum1/1
  clip 2/1 -> Sum1/2

== system vienna_rectifier/afe_dq_mod1/AFE_control/afe_control/current_ctrl/dq_vector_pi/vector lenght ==
  md : Inport
  mq : Inport  Port=2
  Math Function : Math  Operator=magnitude^2  SignedPower=on
  Math Function1 : Math  Operator=magnitude^2  SignedPower=on
  Math Function2 : Math  Operator=reciprocal  SignedPower=on
  Sqrt : Sqrt
  Sum5 : Sum  SaturateOnIntegerOverflow=on
  m_1 : Outport  VectorParamsAs1DForOutWhenUnconnected=off
  m : Outport  Port=2  VectorParamsAs1DForOutWhenUnconnected=off
  wires:
  Sqrt/1 -> m/1, Math Function2/1
  mq/1 -> Math Function1/1
  Math Function1/1 -> Sum5/2
  Math Function/1 -> Sum5/1
  Sum5/1 -> Sqrt/1
  Math Function2/1 -> m_1/1
  md/1 -> Math Function/1

== system vienna_rectifier/afe_dq_mod1/AFE_control/afe_control/current_ctrl/zero_current_ctrl/iz ==
  Demux : Demux  Outputs=3
  Gain : Gain  Gain=1/3
  Sum : Sum  Inputs=+++
  iz : Outport
  wires:
  Sum/1 -> Gain/1
  Demux/1 -> Sum/1  "is_a"
  [isd_abc_pu] -> Demux/1
  Demux/3 -> Sum/3  "is_c"
  Demux/2 -> Sum/2  "is_b"
  Gain/1 -> iz/1
